simulink model "model_new"  (R2023a)
settings: Solver=VariableStepAuto  StartTime=0.0  StopTime=0.5  RelTol=1e-3
model workspace: external: MATLAB File model_new_DataFile.m (data not in the file)
values from neighbouring files (symbols this model uses):
  smiData = struct    [model_new_DataFile.m]
undefined symbols (not defined in the file or in its folder): _, ____, ____16, ____19, ____20, ____3, ____4, ____4X6X3, ____6, ____6X10X3, ____7X11X2, ______, ______1, ______2, ______3_________________________, _______1_________________________2_________________________________航发支架总装, ________, ________1, ________20__1____6, ________6, _________, __________, __________2, __________40160, __________6x16x5, ____________, ____________2, ____________3X1, ______________, ______________1X5, __________________, ___________________, ____________________20__26____4, ____________________25__25____5, __________________SULERCH, ______________A, __________A, __________B, ______A__6, _X2_4E1D6746_X0_, _X2_652F64915EA7_X0_, _X2_7535673A5B8988C5677F_X0_, _X2_8F74627F677F_X0_, _航发支架总装, _默认_sldprt, A25, a__________100, BZ, C, CONNECTOR_5MMCLOSED2PIN_MALE_1, D1, DIP_SWITCH_8PIN_VIC2_1, DYJN, EC, EE, FUS606_REF_1, GE4C, IPOS__________, LAF30, M3________ ... (+34)
libraries: sm_lib x990, nesl_utility x6, simulink x4
(part 13 of 18)

== system model_new/x__25_07_22_V1_STEP_1_RIGID/Subsystem/C_MPU10_20_38_30_STEP_1_RIGID/CHAIN_LINK1_U_C_MPU10_20_38_30_STEP_15_RIGID ==
  ReferenceFrame : sm_lib/Frames and Transforms/Reference Frame
  Solid : sm_lib/Body Elements/File Solid  ExtGeomFileName=CHAIN LINK1 U_C-MPU10-20-38-30.STEP_默认_sldprt.STEP  UnitType=FromFile  ExtGeomFileUnits=m  StepReaderType=HEX  ExportConvexHullGeometry=off  InertiaType=Custom  Mass=smiData.Solid(29).mass  MassUnits=kg  CenterOfMass=smiData.Solid(29).CoM  CenterOfMassUnits=mm  MomentsOfInertia=smiData.Solid(29).MoI  MomentsOfInertiaUnits=kg*mm^2  ProductsOfInertia=smiData.Solid(29).PoI  ProductsOfInertiaUnits=kg*mm^2  BasedOnType=DensityFromFile  Density=1000  DensityUnits=kg/m^3  DoExposeReferenceFrame=on  SerializedFrames=<Frames/>  GraphicType=FromGeometry  MarkerShape=Sphere  MarkerSize=10  GraphicVisPropType=SimpleVisualProperties  GraphicDiffuseColor=smiData.Solid(29).color  GraphicSpecularColor=[0.5 0.5 0.5 1.0]  GraphicAmbientColor=[0.15 0.15 0.15 1.0]  GraphicEmissiveColor=[0.0 0.0 0.0 1.0]  GraphicShininess=75  GraphicOpacity=smiData.Solid(29).opacity
  F : PMIOPort  Side=Left
  connections:
  Solid/RConn1 -- ReferenceFrame/RConn1 -- F/RConn1

== system model_new/x__25_07_22_V1_STEP_1_RIGID/Subsystem/C_MPU10_20_38_30_STEP_1_RIGID/CHAIN_LINK1_U_C_MPU10_20_38_30_STEP_16_RIGID ==
  ReferenceFrame : sm_lib/Frames and Transforms/Reference Frame
  Solid : sm_lib/Body Elements/File Solid  ExtGeomFileName=CHAIN LINK1 U_C-MPU10-20-38-30.STEP_默认_sldprt.STEP  UnitType=FromFile  ExtGeomFileUnits=m  StepReaderType=HEX  ExportConvexHullGeometry=off  InertiaType=Custom  Mass=smiData.Solid(29).mass  MassUnits=kg  CenterOfMass=smiData.Solid(29).CoM  CenterOfMassUnits=mm  MomentsOfInertia=smiData.Solid(29).MoI  MomentsOfInertiaUnits=kg*mm^2  ProductsOfInertia=smiData.Solid(29).PoI  ProductsOfInertiaUnits=kg*mm^2  BasedOnType=DensityFromFile  Density=1000  DensityUnits=kg/m^3  DoExposeReferenceFrame=on  SerializedFrames=<Frames/>  GraphicType=FromGeometry  MarkerShape=Sphere  MarkerSize=10  GraphicVisPropType=SimpleVisualProperties  GraphicDiffuseColor=smiData.Solid(29).color  GraphicSpecularColor=[0.5 0.5 0.5 1.0]  GraphicAmbientColor=[0.15 0.15 0.15 1.0]  GraphicEmissiveColor=[0.0 0.0 0.0 1.0]  GraphicShininess=75  GraphicOpacity=smiData.Solid(29).opacity
  F : PMIOPort  Side=Left
  connections:
  Solid/RConn1 -- ReferenceFrame/RConn1 -- F/RConn1

== system model_new/x__25_07_22_V1_STEP_1_RIGID/Subsystem/C_MPU10_20_38_30_STEP_1_RIGID/CHAIN_LINK1_U_C_MPU10_20_38_30_STEP_17_RIGID ==
  ReferenceFrame : sm_lib/Frames and Transforms/Reference Frame
  Solid : sm_lib/Body Elements/File Solid  ExtGeomFileName=CHAIN LINK1 U_C-MPU10-20-38-30.STEP_默认_sldprt.STEP  UnitType=FromFile  ExtGeomFileUnits=m  StepReaderType=HEX  ExportConvexHullGeometry=off  InertiaType=Custom  Mass=smiData.Solid(29).mass  MassUnits=kg  CenterOfMass=smiData.Solid(29).CoM  CenterOfMassUnits=mm  MomentsOfInertia=smiData.Solid(29).MoI  MomentsOfInertiaUnits=kg*mm^2  ProductsOfInertia=smiData.Solid(29).PoI  ProductsOfInertiaUnits=kg*mm^2  BasedOnType=DensityFromFile  Density=1000  DensityUnits=kg/m^3  DoExposeReferenceFrame=on  SerializedFrames=<Frames/>  GraphicType=FromGeometry  MarkerShape=Sphere  MarkerSize=10  GraphicVisPropType=SimpleVisualProperties  GraphicDiffuseColor=smiData.Solid(29).color  GraphicSpecularColor=[0.5 0.5 0.5 1.0]  GraphicAmbientColor=[0.15 0.15 0.15 1.0]  GraphicEmissiveColor=[0.0 0.0 0.0 1.0]  GraphicShininess=75  GraphicOpacity=smiData.Solid(29).opacity
  F : PMIOPort  Side=Left
  connections:
  Solid/RConn1 -- ReferenceFrame/RConn1 -- F/RConn1

== system model_new/x__25_07_22_V1_STEP_1_RIGID/Subsystem/C_MPU10_20_38_30_STEP_1_RIGID/CHAIN_LINK1_U_C_MPU10_20_38_30_STEP_18_RIGID ==
  ReferenceFrame : sm_lib/Frames and Transforms/Reference Frame
  Solid : sm_lib/Body Elements/File Solid  ExtGeomFileName=CHAIN LINK1 U_C-MPU10-20-38-30.STEP_默认_sldprt.STEP  UnitType=FromFile  ExtGeomFileUnits=m  StepReaderType=HEX  ExportConvexHullGeometry=off  InertiaType=Custom  Mass=smiData.Solid(29).mass  MassUnits=kg  CenterOfMass=smiData.Solid(29).CoM  CenterOfMassUnits=mm  MomentsOfInertia=smiData.Solid(29).MoI  MomentsOfInertiaUnits=kg*mm^2  ProductsOfInertia=smiData.Solid(29).PoI  ProductsOfInertiaUnits=kg*mm^2  BasedOnType=DensityFromFile  Density=1000  DensityUnits=kg/m^3  DoExposeReferenceFrame=on  SerializedFrames=<Frames/>  GraphicType=FromGeometry  MarkerShape=Sphere  MarkerSize=10  GraphicVisPropType=SimpleVisualProperties  GraphicDiffuseColor=smiData.Solid(29).color  GraphicSpecularColor=[0.5 0.5 0.5 1.0]  GraphicAmbientColor=[0.15 0.15 0.15 1.0]  GraphicEmissiveColor=[0.0 0.0 0.0 1.0]  GraphicShininess=75  GraphicOpacity=smiData.Solid(29).opacity
  F : PMIOPort  Side=Left
  connections:
  Solid/RConn1 -- ReferenceFrame/RConn1 -- F/RConn1

== system model_new/x__25_07_22_V1_STEP_1_RIGID/Subsystem/C_MPU10_20_38_30_STEP_1_RIGID/CHAIN_LINK1_U_C_MPU10_20_38_30_STEP_19_RIGID ==
  ReferenceFrame : sm_lib/Frames and Transforms/Reference Frame
  Solid : sm_lib/Body Elements/File Solid  ExtGeomFileName=CHAIN LINK1 U_C-MPU10-20-38-30.STEP_默认_sldprt.STEP  UnitType=FromFile  ExtGeomFileUnits=m  StepReaderType=HEX  ExportConvexHullGeometry=off  InertiaType=Custom  Mass=smiData.Solid(29).mass  MassUnits=kg  CenterOfMass=smiData.Solid(29).CoM  CenterOfMassUnits=mm  MomentsOfInertia=smiData.Solid(29).MoI  MomentsOfInertiaUnits=kg*mm^2  ProductsOfInertia=smiData.Solid(29).PoI  ProductsOfInertiaUnits=kg*mm^2  BasedOnType=DensityFromFile  Density=1000  DensityUnits=kg/m^3  DoExposeReferenceFrame=on  SerializedFrames=<Frames/>  GraphicType=FromGeometry  MarkerShape=Sphere  MarkerSize=10  GraphicVisPropType=SimpleVisualProperties  GraphicDiffuseColor=smiData.Solid(29).color  GraphicSpecularColor=[0.5 0.5 0.5 1.0]  GraphicAmbientColor=[0.15 0.15 0.15 1.0]  GraphicEmissiveColor=[0.0 0.0 0.0 1.0]  GraphicShininess=75  GraphicOpacity=smiData.Solid(29).opacity
  F : PMIOPort  Side=Left
  connections:
  Solid/RConn1 -- ReferenceFrame/RConn1 -- F/RConn1

== system model_new/x__25_07_22_V1_STEP_1_RIGID/Subsystem/C_MPU10_20_38_30_STEP_1_RIGID/CHAIN_LINK1_U_C_MPU10_20_38_30_STEP_1_RIGID ==
  ReferenceFrame : sm_lib/Frames and Transforms/Reference Frame
  Solid : sm_lib/Body Elements/File Solid  ExtGeomFileName=CHAIN LINK1 U_C-MPU10-20-38-30.STEP_默认_sldprt.STEP  UnitType=FromFile  ExtGeomFileUnits=m  StepReaderType=HEX  ExportConvexHullGeometry=off  InertiaType=Custom  Mass=smiData.Solid(29).mass  MassUnits=kg  CenterOfMass=smiData.Solid(29).CoM  CenterOfMassUnits=mm  MomentsOfInertia=smiData.Solid(29).MoI  MomentsOfInertiaUnits=kg*mm^2  ProductsOfInertia=smiData.Solid(29).PoI  ProductsOfInertiaUnits=kg*mm^2  BasedOnType=DensityFromFile  Density=1000  DensityUnits=kg/m^3  DoExposeReferenceFrame=on  SerializedFrames=<Frames/>  GraphicType=FromGeometry  MarkerShape=Sphere  MarkerSize=10  GraphicVisPropType=SimpleVisualProperties  GraphicDiffuseColor=smiData.Solid(29).color  GraphicSpecularColor=[0.5 0.5 0.5 1.0]  GraphicAmbientColor=[0.15 0.15 0.15 1.0]  GraphicEmissiveColor=[0.0 0.0 0.0 1.0]  GraphicShininess=75  GraphicOpacity=smiData.Solid(29).opacity
  F : PMIOPort  Side=Left
  connections:
  Solid/RConn1 -- ReferenceFrame/RConn1 -- F/RConn1

== system model_new/x__25_07_22_V1_STEP_1_RIGID/Subsystem/C_MPU10_20_38_30_STEP_1_RIGID/CHAIN_LINK1_U_C_MPU10_20_38_30_STEP_20_RIGID ==
  ReferenceFrame : sm_lib/Frames and Transforms/Reference Frame
  Solid : sm_lib/Body Elements/File Solid  ExtGeomFileName=CHAIN LINK1 U_C-MPU10-20-38-30.STEP_默认_sldprt.STEP  UnitType=FromFile  ExtGeomFileUnits=m  StepReaderType=HEX  ExportConvexHullGeometry=off  InertiaType=Custom  Mass=smiData.Solid(29).mass  MassUnits=kg  CenterOfMass=smiData.Solid(29).CoM  CenterOfMassUnits=mm  MomentsOfInertia=smiData.Solid(29).MoI  MomentsOfInertiaUnits=kg*mm^2  ProductsOfInertia=smiData.Solid(29).PoI  ProductsOfInertiaUnits=kg*mm^2  BasedOnType=DensityFromFile  Density=1000  DensityUnits=kg/m^3  DoExposeReferenceFrame=on  SerializedFrames=<Frames/>  GraphicType=FromGeometry  MarkerShape=Sphere  MarkerSize=10  GraphicVisPropType=SimpleVisualProperties  GraphicDiffuseColor=smiData.Solid(29).color  GraphicSpecularColor=[0.5 0.5 0.5 1.0]  GraphicAmbientColor=[0.15 0.15 0.15 1.0]  GraphicEmissiveColor=[0.0 0.0 0.0 1.0]  GraphicShininess=75  GraphicOpacity=smiData.Solid(29).opacity
  F : PMIOPort  Side=Left
  connections:
  Solid/RConn1 -- ReferenceFrame/RConn1 -- F/RConn1

== system model_new/x__25_07_22_V1_STEP_1_RIGID/Subsystem/C_MPU10_20_38_30_STEP_1_RIGID/CHAIN_LINK1_U_C_MPU10_20_38_30_STEP_21_RIGID ==
  ReferenceFrame : sm_lib/Frames and Transforms/Reference Frame
  Solid : sm_lib/Body Elements/File Solid  ExtGeomFileName=CHAIN LINK1 U_C-MPU10-20-38-30.STEP_默认_sldprt.STEP  UnitType=FromFile  ExtGeomFileUnits=m  StepReaderType=HEX  ExportConvexHullGeometry=off  InertiaType=Custom  Mass=smiData.Solid(29).mass  MassUnits=kg  CenterOfMass=smiData.Solid(29).CoM  CenterOfMassUnits=mm  MomentsOfInertia=smiData.Solid(29).MoI  MomentsOfInertiaUnits=kg*mm^2  ProductsOfInertia=smiData.Solid(29).PoI  ProductsOfInertiaUnits=kg*mm^2  BasedOnType=DensityFromFile  Density=1000  DensityUnits=kg/m^3  DoExposeReferenceFrame=on  SerializedFrames=<Frames/>  GraphicType=FromGeometry  MarkerShape=Sphere  MarkerSize=10  GraphicVisPropType=SimpleVisualProperties  GraphicDiffuseColor=smiData.Solid(29).color  GraphicSpecularColor=[0.5 0.5 0.5 1.0]  GraphicAmbientColor=[0.15 0.15 0.15 1.0]  GraphicEmissiveColor=[0.0 0.0 0.0 1.0]  GraphicShininess=75  GraphicOpacity=smiData.Solid(29).opacity
  F : PMIOPort  Side=Left
  connections:
  Solid/RConn1 -- ReferenceFrame/RConn1 -- F/RConn1

== system model_new/x__25_07_22_V1_STEP_1_RIGID/Subsystem/C_MPU10_20_38_30_STEP_1_RIGID/CHAIN_LINK1_U_C_MPU10_20_38_30_STEP_22_RIGID ==
  ReferenceFrame : sm_lib/Frames and Transforms/Reference Frame
  Solid : sm_lib/Body Elements/File Solid  ExtGeomFileName=CHAIN LINK1 U_C-MPU10-20-38-30.STEP_默认_sldprt.STEP  UnitType=FromFile  ExtGeomFileUnits=m  StepReaderType=HEX  ExportConvexHullGeometry=off  InertiaType=Custom  Mass=smiData.Solid(29).mass  MassUnits=kg  CenterOfMass=smiData.Solid(29).CoM  CenterOfMassUnits=mm  MomentsOfInertia=smiData.Solid(29).MoI  MomentsOfInertiaUnits=kg*mm^2  ProductsOfInertia=smiData.Solid(29).PoI  ProductsOfInertiaUnits=kg*mm^2  BasedOnType=DensityFromFile  Density=1000  DensityUnits=kg/m^3  DoExposeReferenceFrame=on  SerializedFrames=<Frames/>  GraphicType=FromGeometry  MarkerShape=Sphere  MarkerSize=10  GraphicVisPropType=SimpleVisualProperties  GraphicDiffuseColor=smiData.Solid(29).color  GraphicSpecularColor=[0.5 0.5 0.5 1.0]  GraphicAmbientColor=[0.15 0.15 0.15 1.0]  GraphicEmissiveColor=[0.0 0.0 0.0 1.0]  GraphicShininess=75  GraphicOpacity=smiData.Solid(29).opacity
  F : PMIOPort  Side=Left
  connections:
  Solid/RConn1 -- ReferenceFrame/RConn1 -- F/RConn1

== system model_new/x__25_07_22_V1_STEP_1_RIGID/Subsystem/C_MPU10_20_38_30_STEP_1_RIGID/CHAIN_LINK1_U_C_MPU10_20_38_30_STEP_23_RIGID ==
  ReferenceFrame : sm_lib/Frames and Transforms/Reference Frame
  Solid : sm_lib/Body Elements/File Solid  ExtGeomFileName=CHAIN LINK1 U_C-MPU10-20-38-30.STEP_默认_sldprt.STEP  UnitType=FromFile  ExtGeomFileUnits=m  StepReaderType=HEX  ExportConvexHullGeometry=off  InertiaType=Custom  Mass=smiData.Solid(29).mass  MassUnits=kg  CenterOfMass=smiData.Solid(29).CoM  CenterOfMassUnits=mm  MomentsOfInertia=smiData.Solid(29).MoI  MomentsOfInertiaUnits=kg*mm^2  ProductsOfInertia=smiData.Solid(29).PoI  ProductsOfInertiaUnits=kg*mm^2  BasedOnType=DensityFromFile  Density=1000  DensityUnits=kg/m^3  DoExposeReferenceFrame=on  SerializedFrames=<Frames/>  GraphicType=FromGeometry  MarkerShape=Sphere  MarkerSize=10  GraphicVisPropType=SimpleVisualProperties  GraphicDiffuseColor=smiData.Solid(29).color  GraphicSpecularColor=[0.5 0.5 0.5 1.0]  GraphicAmbientColor=[0.15 0.15 0.15 1.0]  GraphicEmissiveColor=[0.0 0.0 0.0 1.0]  GraphicShininess=75  GraphicOpacity=smiData.Solid(29).opacity
  F : PMIOPort  Side=Left
  connections:
  Solid/RConn1 -- ReferenceFrame/RConn1 -- F/RConn1

== system model_new/x__25_07_22_V1_STEP_1_RIGID/Subsystem/C_MPU10_20_38_30_STEP_1_RIGID/CHAIN_LINK1_U_C_MPU10_20_38_30_STEP_24_RIGID ==
  ReferenceFrame : sm_lib/Frames and Transforms/Reference Frame
  Solid : sm_lib/Body Elements/File Solid  ExtGeomFileName=CHAIN LINK1 U_C-MPU10-20-38-30.STEP_默认_sldprt.STEP  UnitType=FromFile  ExtGeomFileUnits=m  StepReaderType=HEX  ExportConvexHullGeometry=off  InertiaType=Custom  Mass=smiData.Solid(29).mass  MassUnits=kg  CenterOfMass=smiData.Solid(29).CoM  CenterOfMassUnits=mm  MomentsOfInertia=smiData.Solid(29).MoI  MomentsOfInertiaUnits=kg*mm^2  ProductsOfInertia=smiData.Solid(29).PoI  ProductsOfInertiaUnits=kg*mm^2  BasedOnType=DensityFromFile  Density=1000  DensityUnits=kg/m^3  DoExposeReferenceFrame=on  SerializedFrames=<Frames/>  GraphicType=FromGeometry  MarkerShape=Sphere  MarkerSize=10  GraphicVisPropType=SimpleVisualProperties  GraphicDiffuseColor=smiData.Solid(29).color  GraphicSpecularColor=[0.5 0.5 0.5 1.0]  GraphicAmbientColor=[0.15 0.15 0.15 1.0]  GraphicEmissiveColor=[0.0 0.0 0.0 1.0]  GraphicShininess=75  GraphicOpacity=smiData.Solid(29).opacity
  F : PMIOPort  Side=Left
  connections:
  Solid/RConn1 -- ReferenceFrame/RConn1 -- F/RConn1

== system model_new/x__25_07_22_V1_STEP_1_RIGID/Subsystem/C_MPU10_20_38_30_STEP_1_RIGID/CHAIN_LINK1_U_C_MPU10_20_38_30_STEP_25_RIGID ==
  ReferenceFrame : sm_lib/Frames and Transforms/Reference Frame
  Solid : sm_lib/Body Elements/File Solid  ExtGeomFileName=CHAIN LINK1 U_C-MPU10-20-38-30.STEP_默认_sldprt.STEP  UnitType=FromFile  ExtGeomFileUnits=m  StepReaderType=HEX  ExportConvexHullGeometry=off  InertiaType=Custom  Mass=smiData.Solid(29).mass  MassUnits=kg  CenterOfMass=smiData.Solid(29).CoM  CenterOfMassUnits=mm  MomentsOfInertia=smiData.Solid(29).MoI  MomentsOfInertiaUnits=kg*mm^2  ProductsOfInertia=smiData.Solid(29).PoI  ProductsOfInertiaUnits=kg*mm^2  BasedOnType=DensityFromFile  Density=1000  DensityUnits=kg/m^3  DoExposeReferenceFrame=on  SerializedFrames=<Frames/>  GraphicType=FromGeometry  MarkerShape=Sphere  MarkerSize=10  GraphicVisPropType=SimpleVisualProperties  GraphicDiffuseColor=smiData.Solid(29).color  GraphicSpecularColor=[0.5 0.5 0.5 1.0]  GraphicAmbientColor=[0.15 0.15 0.15 1.0]  GraphicEmissiveColor=[0.0 0.0 0.0 1.0]  GraphicShininess=75  GraphicOpacity=smiData.Solid(29).opacity
  F : PMIOPort  Side=Left
  connections:
  Solid/RConn1 -- ReferenceFrame/RConn1 -- F/RConn1

== system model_new/x__25_07_22_V1_STEP_1_RIGID/Subsystem/C_MPU10_20_38_30_STEP_1_RIGID/CHAIN_LINK1_U_C_MPU10_20_38_30_STEP_26_RIGID ==
  ReferenceFrame : sm_lib/Frames and Transforms/Reference Frame
  Solid : sm_lib/Body Elements/File Solid  ExtGeomFileName=CHAIN LINK1 U_C-MPU10-20-38-30.STEP_默认_sldprt.STEP  UnitType=FromFile  ExtGeomFileUnits=m  StepReaderType=HEX  ExportConvexHullGeometry=off  InertiaType=Custom  Mass=smiData.Solid(29).mass  MassUnits=kg  CenterOfMass=smiData.Solid(29).CoM  CenterOfMassUnits=mm  MomentsOfInertia=smiData.Solid(29).MoI  MomentsOfInertiaUnits=kg*mm^2  ProductsOfInertia=smiData.Solid(29).PoI  ProductsOfInertiaUnits=kg*mm^2  BasedOnType=DensityFromFile  Density=1000  DensityUnits=kg/m^3  DoExposeReferenceFrame=on  SerializedFrames=<Frames/>  GraphicType=FromGeometry  MarkerShape=Sphere  MarkerSize=10  GraphicVisPropType=SimpleVisualProperties  GraphicDiffuseColor=smiData.Solid(29).color  GraphicSpecularColor=[0.5 0.5 0.5 1.0]  GraphicAmbientColor=[0.15 0.15 0.15 1.0]  GraphicEmissiveColor=[0.0 0.0 0.0 1.0]  GraphicShininess=75  GraphicOpacity=smiData.Solid(29).opacity
  F : PMIOPort  Side=Left
  connections:
  Solid/RConn1 -- ReferenceFrame/RConn1 -- F/RConn1

== system model_new/x__25_07_22_V1_STEP_1_RIGID/Subsystem/C_MPU10_20_38_30_STEP_1_RIGID/CHAIN_LINK1_U_C_MPU10_20_38_30_STEP_27_RIGID ==
  ReferenceFrame : sm_lib/Frames and Transforms/Reference Frame
  Solid : sm_lib/Body Elements/File Solid  ExtGeomFileName=CHAIN LINK1 U_C-MPU10-20-38-30.STEP_默认_sldprt.STEP  UnitType=FromFile  ExtGeomFileUnits=m  StepReaderType=HEX  ExportConvexHullGeometry=off  InertiaType=Custom  Mass=smiData.Solid(29).mass  MassUnits=kg  CenterOfMass=smiData.Solid(29).CoM  CenterOfMassUnits=mm  MomentsOfInertia=smiData.Solid(29).MoI  MomentsOfInertiaUnits=kg*mm^2  ProductsOfInertia=smiData.Solid(29).PoI  ProductsOfInertiaUnits=kg*mm^2  BasedOnType=DensityFromFile  Density=1000  DensityUnits=kg/m^3  DoExposeReferenceFrame=on  SerializedFrames=<Frames/>  GraphicType=FromGeometry  MarkerShape=Sphere  MarkerSize=10  GraphicVisPropType=SimpleVisualProperties  GraphicDiffuseColor=smiData.Solid(29).color  GraphicSpecularColor=[0.5 0.5 0.5 1.0]  GraphicAmbientColor=[0.15 0.15 0.15 1.0]  GraphicEmissiveColor=[0.0 0.0 0.0 1.0]  GraphicShininess=75  GraphicOpacity=smiData.Solid(29).opacity
  F : PMIOPort  Side=Left
  connections:
  Solid/RConn1 -- ReferenceFrame/RConn1 -- F/RConn1

== system model_new/x__25_07_22_V1_STEP_1_RIGID/Subsystem/C_MPU10_20_38_30_STEP_1_RIGID/CHAIN_LINK1_U_C_MPU10_20_38_30_STEP_28_RIGID ==
  ReferenceFrame : sm_lib/Frames and Transforms/Reference Frame
  Solid : sm_lib/Body Elements/File Solid  ExtGeomFileName=CHAIN LINK1 U_C-MPU10-20-38-30.STEP_默认_sldprt.STEP  UnitType=FromFile  ExtGeomFileUnits=m  StepReaderType=HEX  ExportConvexHullGeometry=off  InertiaType=Custom  Mass=smiData.Solid(29).mass  MassUnits=kg  CenterOfMass=smiData.Solid(29).CoM  CenterOfMassUnits=mm  MomentsOfInertia=smiData.Solid(29).MoI  MomentsOfInertiaUnits=kg*mm^2  ProductsOfInertia=smiData.Solid(29).PoI  ProductsOfInertiaUnits=kg*mm^2  BasedOnType=DensityFromFile  Density=1000  DensityUnits=kg/m^3  DoExposeReferenceFrame=on  SerializedFrames=<Frames/>  GraphicType=FromGeometry  MarkerShape=Sphere  MarkerSize=10  GraphicVisPropType=SimpleVisualProperties  GraphicDiffuseColor=smiData.Solid(29).color  GraphicSpecularColor=[0.5 0.5 0.5 1.0]  GraphicAmbientColor=[0.15 0.15 0.15 1.0]  GraphicEmissiveColor=[0.0 0.0 0.0 1.0]  GraphicShininess=75  GraphicOpacity=smiData.Solid(29).opacity
  F : PMIOPort  Side=Left
  connections:
  Solid/RConn1 -- ReferenceFrame/RConn1 -- F/RConn1

== system model_new/x__25_07_22_V1_STEP_1_RIGID/Subsystem/C_MPU10_20_38_30_STEP_1_RIGID/CHAIN_LINK1_U_C_MPU10_20_38_30_STEP_29_RIGID ==
  ReferenceFrame : sm_lib/Frames and Transforms/Reference Frame
  Solid : sm_lib/Body Elements/File Solid  ExtGeomFileName=CHAIN LINK1 U_C-MPU10-20-38-30.STEP_默认_sldprt.STEP  UnitType=FromFile  ExtGeomFileUnits=m  StepReaderType=HEX  ExportConvexHullGeometry=off  InertiaType=Custom  Mass=smiData.Solid(29).mass  MassUnits=kg  CenterOfMass=smiData.Solid(29).CoM  CenterOfMassUnits=mm  MomentsOfInertia=smiData.Solid(29).MoI  MomentsOfInertiaUnits=kg*mm^2  ProductsOfInertia=smiData.Solid(29).PoI  ProductsOfInertiaUnits=kg*mm^2  BasedOnType=DensityFromFile  Density=1000  DensityUnits=kg/m^3  DoExposeReferenceFrame=on  SerializedFrames=<Frames/>  GraphicType=FromGeometry  MarkerShape=Sphere  MarkerSize=10  GraphicVisPropType=SimpleVisualProperties  GraphicDiffuseColor=smiData.Solid(29).color  GraphicSpecularColor=[0.5 0.5 0.5 1.0]  GraphicAmbientColor=[0.15 0.15 0.15 1.0]  GraphicEmissiveColor=[0.0 0.0 0.0 1.0]  GraphicShininess=75  GraphicOpacity=smiData.Solid(29).opacity
  F : PMIOPort  Side=Left
  connections:
  Solid/RConn1 -- ReferenceFrame/RConn1 -- F/RConn1

== system model_new/x__25_07_22_V1_STEP_1_RIGID/Subsystem/C_MPU10_20_38_30_STEP_1_RIGID/CHAIN_LINK1_U_C_MPU10_20_38_30_STEP_2_RIGID ==
  ReferenceFrame : sm_lib/Frames and Transforms/Reference Frame
  Solid : sm_lib/Body Elements/File Solid  ExtGeomFileName=CHAIN LINK1 U_C-MPU10-20-38-30.STEP_默认_sldprt.STEP  UnitType=FromFile  ExtGeomFileUnits=m  StepReaderType=HEX  ExportConvexHullGeometry=off  InertiaType=Custom  Mass=smiData.Solid(29).mass  MassUnits=kg  CenterOfMass=smiData.Solid(29).CoM  CenterOfMassUnits=mm  MomentsOfInertia=smiData.Solid(29).MoI  MomentsOfInertiaUnits=kg*mm^2  ProductsOfInertia=smiData.Solid(29).PoI  ProductsOfInertiaUnits=kg*mm^2  BasedOnType=DensityFromFile  Density=1000  DensityUnits=kg/m^3  DoExposeReferenceFrame=on  SerializedFrames=<Frames/>  GraphicType=FromGeometry  MarkerShape=Sphere  MarkerSize=10  GraphicVisPropType=SimpleVisualProperties  GraphicDiffuseColor=smiData.Solid(29).color  GraphicSpecularColor=[0.5 0.5 0.5 1.0]  GraphicAmbientColor=[0.15 0.15 0.15 1.0]  GraphicEmissiveColor=[0.0 0.0 0.0 1.0]  GraphicShininess=75  GraphicOpacity=smiData.Solid(29).opacity
  F : PMIOPort  Side=Left
  connections:
  Solid/RConn1 -- ReferenceFrame/RConn1 -- F/RConn1

== system model_new/x__25_07_22_V1_STEP_1_RIGID/Subsystem/C_MPU10_20_38_30_STEP_1_RIGID/CHAIN_LINK1_U_C_MPU10_20_38_30_STEP_30_RIGID ==
  ReferenceFrame : sm_lib/Frames and Transforms/Reference Frame
  Solid : sm_lib/Body Elements/File Solid  ExtGeomFileName=CHAIN LINK1 U_C-MPU10-20-38-30.STEP_默认_sldprt.STEP  UnitType=FromFile  ExtGeomFileUnits=m  StepReaderType=HEX  ExportConvexHullGeometry=off  InertiaType=Custom  Mass=smiData.Solid(29).mass  MassUnits=kg  CenterOfMass=smiData.Solid(29).CoM  CenterOfMassUnits=mm  MomentsOfInertia=smiData.Solid(29).MoI  MomentsOfInertiaUnits=kg*mm^2  ProductsOfInertia=smiData.Solid(29).PoI  ProductsOfInertiaUnits=kg*mm^2  BasedOnType=DensityFromFile  Density=1000  DensityUnits=kg/m^3  DoExposeReferenceFrame=on  SerializedFrames=<Frames/>  GraphicType=FromGeometry  MarkerShape=Sphere  MarkerSize=10  GraphicVisPropType=SimpleVisualProperties  GraphicDiffuseColor=smiData.Solid(29).color  GraphicSpecularColor=[0.5 0.5 0.5 1.0]  GraphicAmbientColor=[0.15 0.15 0.15 1.0]  GraphicEmissiveColor=[0.0 0.0 0.0 1.0]  GraphicShininess=75  GraphicOpacity=smiData.Solid(29).opacity
  F : PMIOPort  Side=Left
  connections:
  Solid/RConn1 -- ReferenceFrame/RConn1 -- F/RConn1

== system model_new/x__25_07_22_V1_STEP_1_RIGID/Subsystem/C_MPU10_20_38_30_STEP_1_RIGID/CHAIN_LINK1_U_C_MPU10_20_38_30_STEP_3_RIGID ==
  ReferenceFrame : sm_lib/Frames and Transforms/Reference Frame
  Solid : sm_lib/Body Elements/File Solid  ExtGeomFileName=CHAIN LINK1 U_C-MPU10-20-38-30.STEP_默认_sldprt.STEP  UnitType=FromFile  ExtGeomFileUnits=m  StepReaderType=HEX  ExportConvexHullGeometry=off  InertiaType=Custom  Mass=smiData.Solid(29).mass  MassUnits=kg  CenterOfMass=smiData.Solid(29).CoM  CenterOfMassUnits=mm  MomentsOfInertia=smiData.Solid(29).MoI  MomentsOfInertiaUnits=kg*mm^2  ProductsOfInertia=smiData.Solid(29).PoI  ProductsOfInertiaUnits=kg*mm^2  BasedOnType=DensityFromFile  Density=1000  DensityUnits=kg/m^3  DoExposeReferenceFrame=on  SerializedFrames=<Frames/>  GraphicType=FromGeometry  MarkerShape=Sphere  MarkerSize=10  GraphicVisPropType=SimpleVisualProperties  GraphicDiffuseColor=smiData.Solid(29).color  GraphicSpecularColor=[0.5 0.5 0.5 1.0]  GraphicAmbientColor=[0.15 0.15 0.15 1.0]  GraphicEmissiveColor=[0.0 0.0 0.0 1.0]  GraphicShininess=75  GraphicOpacity=smiData.Solid(29).opacity
  F : PMIOPort  Side=Left
  connections:
  Solid/RConn1 -- ReferenceFrame/RConn1 -- F/RConn1

== system model_new/x__25_07_22_V1_STEP_1_RIGID/Subsystem/C_MPU10_20_38_30_STEP_1_RIGID/CHAIN_LINK1_U_C_MPU10_20_38_30_STEP_4_RIGID ==
  ReferenceFrame : sm_lib/Frames and Transforms/Reference Frame
  Solid : sm_lib/Body Elements/File Solid  ExtGeomFileName=CHAIN LINK1 U_C-MPU10-20-38-30.STEP_默认_sldprt.STEP  UnitType=FromFile  ExtGeomFileUnits=m  StepReaderType=HEX  ExportConvexHullGeometry=off  InertiaType=Custom  Mass=smiData.Solid(29).mass  MassUnits=kg  CenterOfMass=smiData.Solid(29).CoM  CenterOfMassUnits=mm  MomentsOfInertia=smiData.Solid(29).MoI  MomentsOfInertiaUnits=kg*mm^2  ProductsOfInertia=smiData.Solid(29).PoI  ProductsOfInertiaUnits=kg*mm^2  BasedOnType=DensityFromFile  Density=1000  DensityUnits=kg/m^3  DoExposeReferenceFrame=on  SerializedFrames=<Frames/>  GraphicType=FromGeometry  MarkerShape=Sphere  MarkerSize=10  GraphicVisPropType=SimpleVisualProperties  GraphicDiffuseColor=smiData.Solid(29).color  GraphicSpecularColor=[0.5 0.5 0.5 1.0]  GraphicAmbientColor=[0.15 0.15 0.15 1.0]  GraphicEmissiveColor=[0.0 0.0 0.0 1.0]  GraphicShininess=75  GraphicOpacity=smiData.Solid(29).opacity
  F : PMIOPort  Side=Left
  connections:
  Solid/RConn1 -- ReferenceFrame/RConn1 -- F/RConn1

== system model_new/x__25_07_22_V1_STEP_1_RIGID/Subsystem/C_MPU10_20_38_30_STEP_1_RIGID/CHAIN_LINK1_U_C_MPU10_20_38_30_STEP_5_RIGID ==
  ReferenceFrame : sm_lib/Frames and Transforms/Reference Frame
  Solid : sm_lib/Body Elements/File Solid  ExtGeomFileName=CHAIN LINK1 U_C-MPU10-20-38-30.STEP_默认_sldprt.STEP  UnitType=FromFile  ExtGeomFileUnits=m  StepReaderType=HEX  ExportConvexHullGeometry=off  InertiaType=Custom  Mass=smiData.Solid(29).mass  MassUnits=kg  CenterOfMass=smiData.Solid(29).CoM  CenterOfMassUnits=mm  MomentsOfInertia=smiData.Solid(29).MoI  MomentsOfInertiaUnits=kg*mm^2  ProductsOfInertia=smiData.Solid(29).PoI  ProductsOfInertiaUnits=kg*mm^2  BasedOnType=DensityFromFile  Density=1000  DensityUnits=kg/m^3  DoExposeReferenceFrame=on  SerializedFrames=<Frames/>  GraphicType=FromGeometry  MarkerShape=Sphere  MarkerSize=10  GraphicVisPropType=SimpleVisualProperties  GraphicDiffuseColor=smiData.Solid(29).color  GraphicSpecularColor=[0.5 0.5 0.5 1.0]  GraphicAmbientColor=[0.15 0.15 0.15 1.0]  GraphicEmissiveColor=[0.0 0.0 0.0 1.0]  GraphicShininess=75  GraphicOpacity=smiData.Solid(29).opacity
  F : PMIOPort  Side=Left
  connections:
  Solid/RConn1 -- ReferenceFrame/RConn1 -- F/RConn1

== system model_new/x__25_07_22_V1_STEP_1_RIGID/Subsystem/C_MPU10_20_38_30_STEP_1_RIGID/CHAIN_LINK1_U_C_MPU10_20_38_30_STEP_6_RIGID ==
  ReferenceFrame : sm_lib/Frames and Transforms/Reference Frame
  Solid : sm_lib/Body Elements/File Solid  ExtGeomFileName=CHAIN LINK1 U_C-MPU10-20-38-30.STEP_默认_sldprt.STEP  UnitType=FromFile  ExtGeomFileUnits=m  StepReaderType=HEX  ExportConvexHullGeometry=off  InertiaType=Custom  Mass=smiData.Solid(29).mass  MassUnits=kg  CenterOfMass=smiData.Solid(29).CoM  CenterOfMassUnits=mm  MomentsOfInertia=smiData.Solid(29).MoI  MomentsOfInertiaUnits=kg*mm^2  ProductsOfInertia=smiData.Solid(29).PoI  ProductsOfInertiaUnits=kg*mm^2  BasedOnType=DensityFromFile  Density=1000  DensityUnits=kg/m^3  DoExposeReferenceFrame=on  SerializedFrames=<Frames/>  GraphicType=FromGeometry  MarkerShape=Sphere  MarkerSize=10  GraphicVisPropType=SimpleVisualProperties  GraphicDiffuseColor=smiData.Solid(29).color  GraphicSpecularColor=[0.5 0.5 0.5 1.0]  GraphicAmbientColor=[0.15 0.15 0.15 1.0]  GraphicEmissiveColor=[0.0 0.0 0.0 1.0]  GraphicShininess=75  GraphicOpacity=smiData.Solid(29).opacity
  F : PMIOPort  Side=Left
  connections:
  Solid/RConn1 -- ReferenceFrame/RConn1 -- F/RConn1

== system model_new/x__25_07_22_V1_STEP_1_RIGID/Subsystem/C_MPU10_20_38_30_STEP_1_RIGID/CHAIN_LINK1_U_C_MPU10_20_38_30_STEP_7_RIGID ==
  ReferenceFrame : sm_lib/Frames and Transforms/Reference Frame
  Solid : sm_lib/Body Elements/File Solid  ExtGeomFileName=CHAIN LINK1 U_C-MPU10-20-38-30.STEP_默认_sldprt.STEP  UnitType=FromFile  ExtGeomFileUnits=m  StepReaderType=HEX  ExportConvexHullGeometry=off  InertiaType=Custom  Mass=smiData.Solid(29).mass  MassUnits=kg  CenterOfMass=smiData.Solid(29).CoM  CenterOfMassUnits=mm  MomentsOfInertia=smiData.Solid(29).MoI  MomentsOfInertiaUnits=kg*mm^2  ProductsOfInertia=smiData.Solid(29).PoI  ProductsOfInertiaUnits=kg*mm^2  BasedOnType=DensityFromFile  Density=1000  DensityUnits=kg/m^3  DoExposeReferenceFrame=on  SerializedFrames=<Frames/>  GraphicType=FromGeometry  MarkerShape=Sphere  MarkerSize=10  GraphicVisPropType=SimpleVisualProperties  GraphicDiffuseColor=smiData.Solid(29).color  GraphicSpecularColor=[0.5 0.5 0.5 1.0]  GraphicAmbientColor=[0.15 0.15 0.15 1.0]  GraphicEmissiveColor=[0.0 0.0 0.0 1.0]  GraphicShininess=75  GraphicOpacity=smiData.Solid(29).opacity
  F : PMIOPort  Side=Left
  connections:
  Solid/RConn1 -- ReferenceFrame/RConn1 -- F/RConn1

== system model_new/x__25_07_22_V1_STEP_1_RIGID/Subsystem/C_MPU10_20_38_30_STEP_1_RIGID/CHAIN_LINK1_U_C_MPU10_20_38_30_STEP_8_RIGID ==
  ReferenceFrame : sm_lib/Frames and Transforms/Reference Frame
  Solid : sm_lib/Body Elements/File Solid  ExtGeomFileName=CHAIN LINK1 U_C-MPU10-20-38-30.STEP_默认_sldprt.STEP  UnitType=FromFile  ExtGeomFileUnits=m  StepReaderType=HEX  ExportConvexHullGeometry=off  InertiaType=Custom  Mass=smiData.Solid(29).mass  MassUnits=kg  CenterOfMass=smiData.Solid(29).CoM  CenterOfMassUnits=mm  MomentsOfInertia=smiData.Solid(29).MoI  MomentsOfInertiaUnits=kg*mm^2  ProductsOfInertia=smiData.Solid(29).PoI  ProductsOfInertiaUnits=kg*mm^2  BasedOnType=DensityFromFile  Density=1000  DensityUnits=kg/m^3  DoExposeReferenceFrame=on  SerializedFrames=<Frames/>  GraphicType=FromGeometry  MarkerShape=Sphere  MarkerSize=10  GraphicVisPropType=SimpleVisualProperties  GraphicDiffuseColor=smiData.Solid(29).color  GraphicSpecularColor=[0.5 0.5 0.5 1.0]  GraphicAmbientColor=[0.15 0.15 0.15 1.0]  GraphicEmissiveColor=[0.0 0.0 0.0 1.0]  GraphicShininess=75  GraphicOpacity=smiData.Solid(29).opacity
  F : PMIOPort  Side=Left
  connections:
  Solid/RConn1 -- ReferenceFrame/RConn1 -- F/RConn1

== system model_new/x__25_07_22_V1_STEP_1_RIGID/Subsystem/C_MPU10_20_38_30_STEP_1_RIGID/CHAIN_LINK1_U_C_MPU10_20_38_30_STEP_9_RIGID ==
  ReferenceFrame : sm_lib/Frames and Transforms/Reference Frame
  Solid : sm_lib/Body Elements/File Solid  ExtGeomFileName=CHAIN LINK1 U_C-MPU10-20-38-30.STEP_默认_sldprt.STEP  UnitType=FromFile  ExtGeomFileUnits=m  StepReaderType=HEX  ExportConvexHullGeometry=off  InertiaType=Custom  Mass=smiData.Solid(29).mass  MassUnits=kg  CenterOfMass=smiData.Solid(29).CoM  CenterOfMassUnits=mm  MomentsOfInertia=smiData.Solid(29).MoI  MomentsOfInertiaUnits=kg*mm^2  ProductsOfInertia=smiData.Solid(29).PoI  ProductsOfInertiaUnits=kg*mm^2  BasedOnType=DensityFromFile  Density=1000  DensityUnits=kg/m^3  DoExposeReferenceFrame=on  SerializedFrames=<Frames/>  GraphicType=FromGeometry  MarkerShape=Sphere  MarkerSize=10  GraphicVisPropType=SimpleVisualProperties  GraphicDiffuseColor=smiData.Solid(29).color  GraphicSpecularColor=[0.5 0.5 0.5 1.0]  GraphicAmbientColor=[0.15 0.15 0.15 1.0]  GraphicEmissiveColor=[0.0 0.0 0.0 1.0]  GraphicShininess=75  GraphicOpacity=smiData.Solid(29).opacity
  F : PMIOPort  Side=Left
  connections:
  Solid/RConn1 -- ReferenceFrame/RConn1 -- F/RConn1

== system model_new/x__25_07_22_V1_STEP_1_RIGID/Subsystem/x__25_07_22_V1_STEP_1_RIGID1/CL3J_EC503_3D_25_07_22_V1_STEP_1_RIGID ==
  CONNECTOR_5MMCLOSED2PIN_MALE_125_07_22_V1_STEP_1_RIGID : Subsystem
  PCB_ASM_4_ASM25_07_22_V1_STEP_1_RIGID : Subsystem
  ReferenceFrame : sm_lib/Frames and Transforms/Reference Frame
  Transform : sm_lib/Frames and Transforms/Rigid Transform  TranslationMethod=Cartesian  TranslationStandardOffset=0  TranslationStandardOffsetUnits=m  TranslationStandardAxis=+Z  TranslationCartesianOffset=smiData.RigidTransform(172).translation  TranslationCartesianOffsetUnits=mm  TranslationROffset=0  TranslationROffsetUnits=m  TranslationZOffset=0  TranslationZOffsetUnits=m  TranslationThetaOffset=0  TranslationThetaOffsetUnits=deg  RotationMethod=ArbitraryAxis  RotationAngleUnits=rad  RotationStandardAxis=+Z  RotationAngle=smiData.RigidTransform(172).angle  RotationArbitraryAxis=smiData.RigidTransform(172).axis  FollAlignAxisA=+X  BaseAlignAxisA=+Y  FollAlignAxisB=+Y  BaseAlignAxisB=+Z  RotationSequenceAxes=FollowerAxes  RotationSequence=XYX  RotationSequenceAngles=[0 0 0]  RotationSequenceAnglesUnits=deg  RotationMatrix=[1 0 0; 0 1 0; 0 0 1]  Quaternion=[1 0 0 0]
  Transform1 : sm_lib/Frames and Transforms/Rigid Transform  TranslationMethod=Cartesian  TranslationStandardOffset=0  TranslationStandardOffsetUnits=m  TranslationStandardAxis=+Z  TranslationCartesianOffset=smiData.RigidTransform(197).translation  TranslationCartesianOffsetUnits=mm  TranslationROffset=0  TranslationROffsetUnits=m  TranslationZOffset=0  TranslationZOffsetUnits=m  TranslationThetaOffset=0  TranslationThetaOffsetUnits=deg  RotationMethod=ArbitraryAxis  RotationAngleUnits=rad  RotationStandardAxis=+Z  RotationAngle=smiData.RigidTransform(197).angle  RotationArbitraryAxis=smiData.RigidTransform(197).axis  FollAlignAxisA=+X  BaseAlignAxisA=+Y  FollAlignAxisB=+Y  BaseAlignAxisB=+Z  RotationSequenceAxes=FollowerAxes  RotationSequence=XYX  RotationSequenceAngles=[0 0 0]  RotationSequenceAnglesUnits=deg  RotationMatrix=[1 0 0; 0 1 0; 0 0 1]  Quaternion=[1 0 0 0]
  Transform2 : sm_lib/Frames and Transforms/Rigid Transform  TranslationMethod=Cartesian  TranslationStandardOffset=0  TranslationStandardOffsetUnits=m  TranslationStandardAxis=+Z  TranslationCartesianOffset=smiData.RigidTransform(198).translation  TranslationCartesianOffsetUnits=mm  TranslationROffset=0  TranslationROffsetUnits=m  TranslationZOffset=0  TranslationZOffsetUnits=m  TranslationThetaOffset=0  TranslationThetaOffsetUnits=deg  RotationMethod=ArbitraryAxis  RotationAngleUnits=rad  RotationStandardAxis=+Z  RotationAngle=smiData.RigidTransform(198).angle  RotationArbitraryAxis=smiData.RigidTransform(198).axis  FollAlignAxisA=+X  BaseAlignAxisA=+Y  FollAlignAxisB=+Y  BaseAlignAxisB=+Z  RotationSequenceAxes=FollowerAxes  RotationSequence=XYX  RotationSequenceAngles=[0 0 0]  RotationSequenceAnglesUnits=deg  RotationMatrix=[1 0 0; 0 1 0; 0 0 1]  Quaternion=[1 0 0 0]
  Transform3 : sm_lib/Frames and Transforms/Rigid Transform  TranslationMethod=Cartesian  TranslationStandardOffset=0  TranslationStandardOffsetUnits=m  TranslationStandardAxis=+Z  TranslationCartesianOffset=smiData.RigidTransform(199).translation  TranslationCartesianOffsetUnits=mm  TranslationROffset=0  TranslationROffsetUnits=m  TranslationZOffset=0  TranslationZOffsetUnits=m  TranslationThetaOffset=0  TranslationThetaOffsetUnits=deg  RotationMethod=ArbitraryAxis  RotationAngleUnits=rad  RotationStandardAxis=+Z  RotationAngle=smiData.RigidTransform(199).angle  RotationArbitraryAxis=smiData.RigidTransform(199).axis  FollAlignAxisA=+X  BaseAlignAxisA=+Y  FollAlignAxisB=+Y  BaseAlignAxisB=+Z  RotationSequenceAxes=FollowerAxes  RotationSequence=XYX  RotationSequenceAngles=[0 0 0]  RotationSequenceAnglesUnits=deg  RotationMatrix=[1 0 0; 0 1 0; 0 0 1]  Quaternion=[1 0 0 0]
  x1_425_07_22_V1_STEP_1_RIGID : Subsystem
  x2_1125_07_22_V1_STEP_1_RIGID : Subsystem
  F : PMIOPort  Side=Right
  connections:
  CONNECTOR_5MMCLOSED2PIN_MALE_125_07_22_V1_STEP_1_RIGID/LConn1 -- Transform/RConn1
  Transform1/RConn1 -- x1_425_07_22_V1_STEP_1_RIGID/LConn1
  Transform2/RConn1 -- x2_1125_07_22_V1_STEP_1_RIGID/LConn1
  ReferenceFrame/RConn1 -- PCB_ASM_4_ASM25_07_22_V1_STEP_1_RIGID/RConn1 -- Transform/LConn1 -- Transform1/LConn1 -- Transform2/LConn1 -- Transform3/RConn1
  Transform3/LConn1 -- F/RConn1

== system model_new/x__25_07_22_V1_STEP_1_RIGID/Subsystem/x__25_07_22_V1_STEP_1_RIGID1/M3_25_07_22_V1_STEP_1_RIGID ==
  ReferenceFrame : sm_lib/Frames and Transforms/Reference Frame
  Solid : sm_lib/Body Elements/File Solid  ExtGeomFileName=M3________(25.07.22)-V1.STEP_默认_sldprt.STEP  UnitType=FromFile  ExtGeomFileUnits=m  StepReaderType=HEX  ExportConvexHullGeometry=off  InertiaType=Custom  Mass=smiData.Solid(108).mass  MassUnits=kg  CenterOfMass=smiData.Solid(108).CoM  CenterOfMassUnits=mm  MomentsOfInertia=smiData.Solid(108).MoI  MomentsOfInertiaUnits=kg*mm^2  ProductsOfInertia=smiData.Solid(108).PoI  ProductsOfInertiaUnits=kg*mm^2  BasedOnType=DensityFromFile  Density=1000  DensityUnits=kg/m^3  DoExposeReferenceFrame=on  SerializedFrames=<Frames/>  GraphicType=FromGeometry  MarkerShape=Sphere  MarkerSize=10  GraphicVisPropType=SimpleVisualProperties  GraphicDiffuseColor=smiData.Solid(108).color  GraphicSpecularColor=[0.5 0.5 0.5 1.0]  GraphicAmbientColor=[0.15 0.15 0.15 1.0]  GraphicEmissiveColor=[0.0 0.0 0.0 1.0]  GraphicShininess=75  GraphicOpacity=smiData.Solid(108).opacity
  F : PMIOPort  Side=Left
  connections:
  Solid/RConn1 -- ReferenceFrame/RConn1 -- F/RConn1

== system model_new/x__25_07_22_V1_STEP_1_RIGID/Subsystem/x__25_07_22_V1_STEP_1_RIGID1/M3_25_07_22_V1_STEP_2_RIGID ==
  ReferenceFrame : sm_lib/Frames and Transforms/Reference Frame
  Solid : sm_lib/Body Elements/File Solid  ExtGeomFileName=M3________(25.07.22)-V1.STEP_默认_sldprt.STEP  UnitType=FromFile  ExtGeomFileUnits=m  StepReaderType=HEX  ExportConvexHullGeometry=off  InertiaType=Custom  Mass=smiData.Solid(108).mass  MassUnits=kg  CenterOfMass=smiData.Solid(108).CoM  CenterOfMassUnits=mm  MomentsOfInertia=smiData.Solid(108).MoI  MomentsOfInertiaUnits=kg*mm^2  ProductsOfInertia=smiData.Solid(108).PoI  ProductsOfInertiaUnits=kg*mm^2  BasedOnType=DensityFromFile  Density=1000  DensityUnits=kg/m^3  DoExposeReferenceFrame=on  SerializedFrames=<Frames/>  GraphicType=FromGeometry  MarkerShape=Sphere  MarkerSize=10  GraphicVisPropType=SimpleVisualProperties  GraphicDiffuseColor=smiData.Solid(108).color  GraphicSpecularColor=[0.5 0.5 0.5 1.0]  GraphicAmbientColor=[0.15 0.15 0.15 1.0]  GraphicEmissiveColor=[0.0 0.0 0.0 1.0]  GraphicShininess=75  GraphicOpacity=smiData.Solid(108).opacity
  F : PMIOPort  Side=Left
  connections:
  Solid/RConn1 -- ReferenceFrame/RConn1 -- F/RConn1

== system model_new/x__25_07_22_V1_STEP_1_RIGID/Subsystem/x__25_07_22_V1_STEP_1_RIGID1/MGR15_temp_125_07_22_V1_STEP_1_RIGID ==
  ReferenceFrame : sm_lib/Frames and Transforms/Reference Frame
  Solid : sm_lib/Body Elements/File Solid  ExtGeomFileName=MGR15_temp-1(25.07.22)-V1.STEP_默认_sldprt.STEP  UnitType=FromFile  ExtGeomFileUnits=m  StepReaderType=HEX  ExportConvexHullGeometry=off  InertiaType=Custom  Mass=smiData.Solid(107).mass  MassUnits=kg  CenterOfMass=smiData.Solid(107).CoM  CenterOfMassUnits=mm  MomentsOfInertia=smiData.Solid(107).MoI  MomentsOfInertiaUnits=kg*mm^2  ProductsOfInertia=smiData.Solid(107).PoI  ProductsOfInertiaUnits=kg*mm^2  BasedOnType=DensityFromFile  Density=1000  DensityUnits=kg/m^3  DoExposeReferenceFrame=on  SerializedFrames=<Frames/>  GraphicType=FromGeometry  MarkerShape=Sphere  MarkerSize=10  GraphicVisPropType=SimpleVisualProperties  GraphicDiffuseColor=smiData.Solid(107).color  GraphicSpecularColor=[0.5 0.5 0.5 1.0]  GraphicAmbientColor=[0.15 0.15 0.15 1.0]  GraphicEmissiveColor=[0.0 0.0 0.0 1.0]  GraphicShininess=75  GraphicOpacity=smiData.Solid(107).opacity
  F : PMIOPort  Side=Left
  connections:
  Solid/RConn1 -- ReferenceFrame/RConn1 -- F/RConn1

== system model_new/x__25_07_22_V1_STEP_1_RIGID/Subsystem/x__25_07_22_V1_STEP_1_RIGID1/MGR15_temp_125_07_22_V1_STEP_2_RIGID ==
  ReferenceFrame : sm_lib/Frames and Transforms/Reference Frame
  Solid : sm_lib/Body Elements/File Solid  ExtGeomFileName=MGR15_temp-1(25.07.22)-V1.STEP_默认_sldprt.STEP  UnitType=FromFile  ExtGeomFileUnits=m  StepReaderType=HEX  ExportConvexHullGeometry=off  InertiaType=Custom  Mass=smiData.Solid(107).mass  MassUnits=kg  CenterOfMass=smiData.Solid(107).CoM  CenterOfMassUnits=mm  MomentsOfInertia=smiData.Solid(107).MoI  MomentsOfInertiaUnits=kg*mm^2  ProductsOfInertia=smiData.Solid(107).PoI  ProductsOfInertiaUnits=kg*mm^2  BasedOnType=DensityFromFile  Density=1000  DensityUnits=kg/m^3  DoExposeReferenceFrame=on  SerializedFrames=<Frames/>  GraphicType=FromGeometry  MarkerShape=Sphere  MarkerSize=10  GraphicVisPropType=SimpleVisualProperties  GraphicDiffuseColor=smiData.Solid(107).color  GraphicSpecularColor=[0.5 0.5 0.5 1.0]  GraphicAmbientColor=[0.15 0.15 0.15 1.0]  GraphicEmissiveColor=[0.0 0.0 0.0 1.0]  GraphicShininess=75  GraphicOpacity=smiData.Solid(107).opacity
  F : PMIOPort  Side=Left
  connections:
  Solid/RConn1 -- ReferenceFrame/RConn1 -- F/RConn1
